simulink model "g1_centroidal_planner"  (R2025b)
settings: Solver=FixedStepDiscrete  StartTime=0.0  StopTime=0.05  FixedStep=0.002  RelTol=1e-3
model workspace (MAT data in the model file):
  accelerationKd = [0; 0; 0; 0; 0; 0; 0; 0; 0; 0; 0; 0; 0; 0; 0; 0; 0; 0; 0; 0; 0; 0; 0]
  accelerationKp = [0; 0; 0; 0; 0; 0; 0; 0; 0; 0; 0; 0; 0; 0; 0; 0; 0; 0; 0; 0; 0; 0; 0]
  g1_mpc_joint_indices = [4 5 6 7 1 2 17 18 19 20 14 15 29 28 27 8 9 10 3 21 22 23 16]
values from neighbouring files (symbols this model uses):
  g1_kd = 10.0 10.0 10.0 10.0 10.0 10.0 10.0 10.0 10.0 10.0 1.0 1.0 1.0 10.0 10.0 10.0 10.0 10.0 10.0 10.0 10.0 10.0 10.0 1.0 1.0 1.0 10.0 10.0 10.0    [g1_data.sldd]
  g1_kp = 1200.0 1200.0 1200.0 1200.0 1200.0 1200.0 1200.0 1200.0 1200.0 1200.0 100.0 100.0 100.0 1200.0 1200.0 1200.0 1200.0 1200.0 1200.0 1200.0 1200.0 1200.0 1200.0 100.0 100.0 100.0 1200.0 1200.0 1200.0    [g1_data.sldd]
  g1_mpc_to_plant = 0.0 0.0 0.0 1.0 0.0 0.0 0.0 0.0 0.0 0.0 0.0 0.0 0.0 0.0 0.0 0.0 0.0 0.0 0.0 0.0 0.0 0.0 0.0 0.0 0.0 0.0 0.0 0.0 0.0 0.0 0.0 0.0 0.0 1.0 0.0 0.0 0.0 0.0 0.0 0.0 0.0 0.0 0.0 0.0 0.0 0.0 0.0 0.0 0.0 0.0 0.0 0.0 0.0 0.0 0.0 0.0 0.0 0.0 0.0 0.0 0.0 0.0 0.0 1.0 0.0 0.0 0.0 0.0 0.0 0.0 0.0 0.0 0.0 0.0 0.0 0.0 0.0 0.0 0.0 0.0 0.0 0.0 0.0 0.0 0.0 0.0 0.0 0.0 0.0 0.0 0.0 0.0 0.0 1.0 0.0 0.0 0.0 0.0 0.0 0.0    [g1_data.sldd]
Description:
  | Centroidal synchronous MPC and policy query followed by independent inverse dynamics using measured q/v. Output: policy72, torque23, action95.
settings Model: DataDictionary=g1_data.sldd  Creator=enoch  LastModifiedBy=enoch

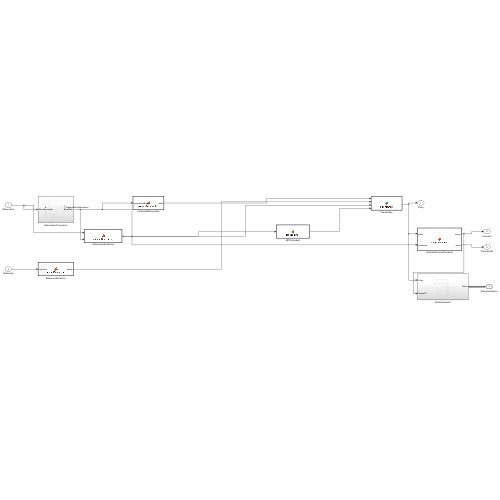
[thumbnail: Simulink's stored preview of the top-level diagram]
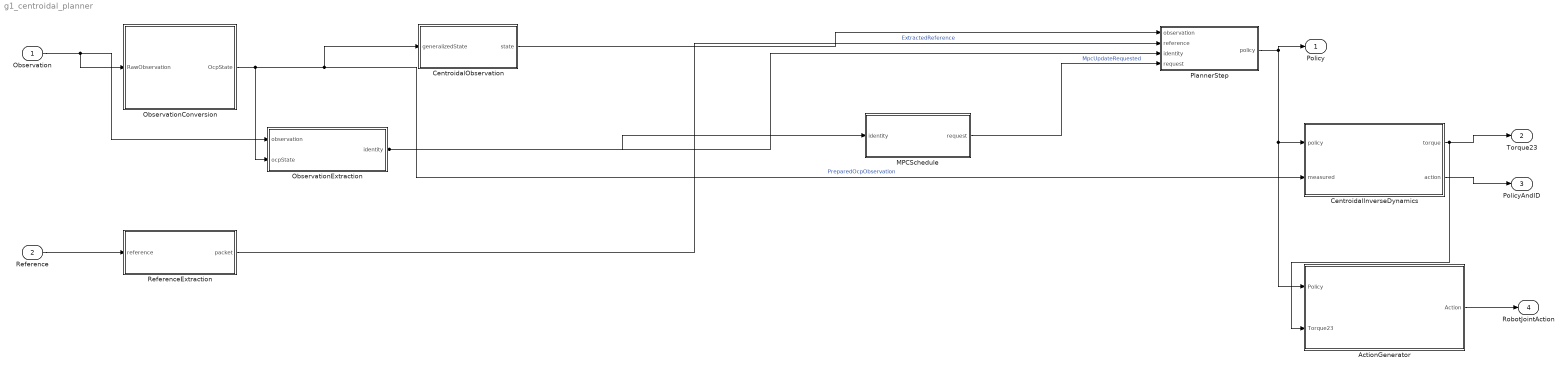
== system g1_centroidal_planner ==
  Observation : Inport  PortDimensions=74  SampleTime=0.002
  Reference : Inport  Port=2  PortDimensions=428  SampleTime=0.002
  ActionGenerator : Subsystem
  CentroidalInverseDynamics : MATLAB Function  TreatAsAtomicUnit=on
  CentroidalObservation : MATLAB Function  TreatAsAtomicUnit=on
  MPCSchedule : MATLAB Function  TreatAsAtomicUnit=on
  ObservationConversion : Subsystem
  ObservationExtraction : MATLAB Function  TreatAsAtomicUnit=on
  PlannerStep : MATLAB Function  TreatAsAtomicUnit=on
  ReferenceExtraction : MATLAB Function  TreatAsAtomicUnit=on
  Policy : Outport  PortDimensions=72
  Torque23 : Outport  Port=2  PortDimensions=23
  PolicyAndID : Outport  Port=3  PortDimensions=95
  RobotJointAction : Outport  Port=4  OutDataTypeStr=Bus: RobotJointAction
  wires:
  Observation/1 -> ObservationConversion/1(RawObservation), ObservationExtraction/1(observation)
  ObservationConversion/1(OcpState) -> CentroidalInverseDynamics/2(measured), CentroidalObservation/1(generalizedState), ObservationExtraction/2(ocpState)  "PreparedOcpObservation"
  Reference/1 -> ReferenceExtraction/1(reference)
  ReferenceExtraction/1(packet) -> PlannerStep/2(reference)  "ExtractedReference"
  CentroidalObservation/1(state) -> PlannerStep/1(observation)
  ObservationExtraction/1(identity) -> PlannerStep/3(identity), MPCSchedule/1(identity)
  MPCSchedule/1(request) -> PlannerStep/4(request)  "MpcUpdateRequested"
  PlannerStep/1(policy) -> Policy/1, ActionGenerator/1(Policy), CentroidalInverseDynamics/1(policy)
  CentroidalInverseDynamics/1(torque) -> Torque23/1, ActionGenerator/2(Torque23)
  CentroidalInverseDynamics/2(action) -> PolicyAndID/1
  ActionGenerator/1(Action) -> RobotJointAction/1

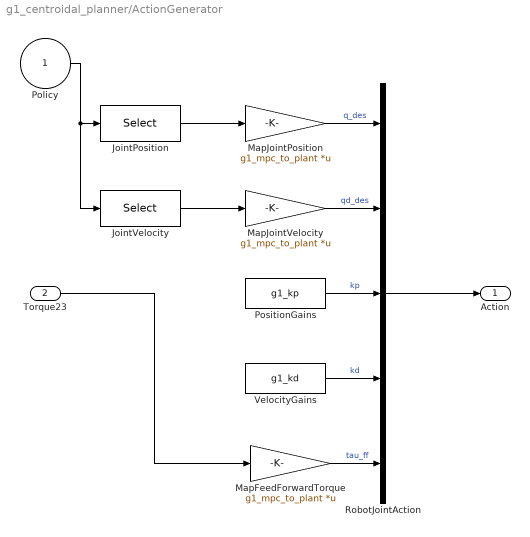
== system g1_centroidal_planner/ActionGenerator ==
  Policy : Inport  PortDimensions=72
  Torque23 : Inport  Port=2  PortDimensions=23
  JointPosition : Selector  InputPortWidth=72  IndexOptions=Index vector (dialog)  Indices=13:35  OutputSizes=1
  JointVelocity : Selector  InputPortWidth=72  IndexOptions=Index vector (dialog)  Indices=48:70  OutputSizes=1
  MapFeedForwardTorque : Gain  Gain=g1_mpc_to_plant  Multiplication=Matrix(K*u)
  MapJointPosition : Gain  Gain=g1_mpc_to_plant  Multiplication=Matrix(K*u)
  MapJointVelocity : Gain  Gain=g1_mpc_to_plant  Multiplication=Matrix(K*u)
  PositionGains : Constant  Value=g1_kp
  RobotJointAction : BusCreator  Inputs=5  OutDataTypeStr=Bus: RobotJointAction  NonVirtualBus=on
  VelocityGains : Constant  Value=g1_kd
  Action : Outport  OutDataTypeStr=Bus: RobotJointAction
  wires:
  MapJointPosition/1 -> RobotJointAction/1  "q_des"
  MapJointVelocity/1 -> RobotJointAction/2  "qd_des"
  PositionGains/1 -> RobotJointAction/3  "kp"
  VelocityGains/1 -> RobotJointAction/4  "kd"
  MapFeedForwardTorque/1 -> RobotJointAction/5  "tau_ff"
  RobotJointAction/1 -> Action/1
  Torque23/1 -> MapFeedForwardTorque/1
  JointVelocity/1 -> MapJointVelocity/1
  JointPosition/1 -> MapJointPosition/1
  Policy/1 -> JointVelocity/1, JointPosition/1

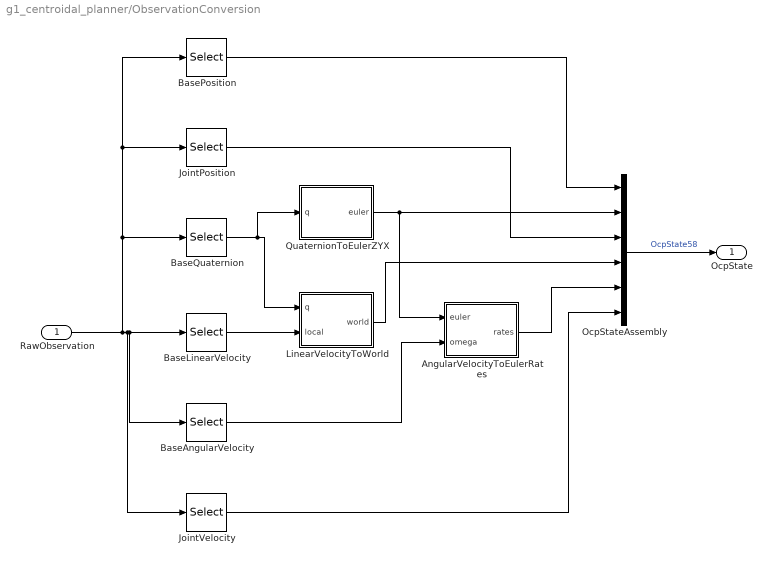
== system g1_centroidal_planner/ObservationConversion ==
  RawObservation : Inport
  AngularVelocityToEulerRates : MATLAB Function  TreatAsAtomicUnit=on
  BaseAngularVelocity : Selector  InputPortWidth=74  IndexOptions=Index vector (dialog)  Indices=12:14  OutputSizes=1
  BaseLinearVelocity : Selector  InputPortWidth=74  IndexOptions=Index vector (dialog)  Indices=9:11  OutputSizes=1
  BasePosition : Selector  InputPortWidth=74  IndexOptions=Index vector (dialog)  Indices=2:4  OutputSizes=1
  BaseQuaternion : Selector  InputPortWidth=74  IndexOptions=Index vector (dialog)  Indices=5:8  OutputSizes=1
  JointPosition : Selector  InputPortWidth=74  IndexOptions=Index vector (dialog)  Indices=14+g1_mpc_joint_indices  OutputSizes=1
  JointVelocity : Selector  InputPortWidth=74  IndexOptions=Index vector (dialog)  Indices=43+g1_mpc_joint_indices  OutputSizes=1
  LinearVelocityToWorld : MATLAB Function  TreatAsAtomicUnit=on
  OcpStateAssembly : Mux  Inputs=6
  QuaternionToEulerZYX : MATLAB Function  TreatAsAtomicUnit=on
  OcpState : Outport
  wires:
  RawObservation/1 -> BaseQuaternion/1, BasePosition/1, JointPosition/1, JointVelocity/1, BaseAngularVelocity/1, BaseLinearVelocity/1
  BaseQuaternion/1 -> LinearVelocityToWorld/1(q), QuaternionToEulerZYX/1(q)
  BasePosition/1 -> OcpStateAssembly/1
  JointPosition/1 -> OcpStateAssembly/3
  JointVelocity/1 -> OcpStateAssembly/6
  OcpStateAssembly/1 -> OcpState/1  "OcpState58"
  BaseLinearVelocity/1 -> LinearVelocityToWorld/2(local)
  QuaternionToEulerZYX/1(euler) -> OcpStateAssembly/2, AngularVelocityToEulerRates/1(euler)
  BaseAngularVelocity/1 -> AngularVelocityToEulerRates/2(omega)
  LinearVelocityToWorld/1(world) -> OcpStateAssembly/4
  AngularVelocityToEulerRates/1(rates) -> OcpStateAssembly/5

== matlab function g1_centroidal_planner/ObservationExtraction ==
  data: observation input; identity output; ocpState input; g1_mpc_joint_indices parameter
function identity = extractObservation(observation, ocpState, g1_mpc_joint_indices)
state=ocpState; indices=g1_mpc_joint_indices;
%EXTRACTOBSERVATION Check observation/state mapping and return tick identity.
%#codegen
% Derived from ObservationExtractionMex.cpp; see licenses/observation_conversion.txt.
assert(isa(observation,'double') && isreal(observation) && ~issparse(observation) && numel(observation)==74,'G1:ObservationExtraction','Invalid observation type or dimension');
assert(isa(state,'double') && isreal(state) && ~issparse(state) && numel(state)==58,'G1:ObservationExtraction','Invalid state type or dimension');
assert(isa(indices,'double') && isreal(indices) && ~issparse(indices) && numel(indices)==23,'G1:ObservationExtraction','Invalid joint index type or dimension');
assert(all(isfinite(observation(:))) && all(isfinite(state(:))),'G1:ObservationExtraction','Nonfinite observation or state');
t=observation(1);
assert(t>=0 && t/.002<=9007199254740992,'G1:ObservationExtraction','Invalid physical time');
tick=round(t/.002); canonical=tick*.002;
assert(abs(t-canonical)<=1e-12,'G1:ObservationExtraction','Raw time exceeds canonical tick tolerance');
assert(observation(4)>=.35 && observation(4)<=1.3,'G1:ObservationExtraction','Base height outside safety envelope');
q=observation(5:8);
pitch=asin(max(-1,min(1,2*(q(1)*q(3)-q(4)*q(2)))));
roll=atan2(2*(q(1)*q(2)+q(3)*q(4)),1-2*(q(2)*q(2)+q(3)*q(3)));
assert(abs(pitch)<=pi/4 && abs(roll)<=pi/4,'G1:ObservationExtraction','Tilt outside safety envelope');
assert(abs(norm(q)-1)<=1e-6,'G1:ObservationExtraction','Quaternion rejected');
for j=1:3
    assert(state(j)==observation(1+j),'G1:ObservationExtraction','OCP position identity mismatch');
end
seen=false(29,1);
for j=1:23
    k=indices(j);
    assert(isfinite(k) && k>=1 && k<=29 && k==floor(k),'G1:ObservationExtraction','Invalid joint index');
    assert(~seen(k),'G1:ObservationExtraction','Duplicate joint index');
    seen(k)=true;
    assert(state(6+j)==observation(14+k) && state(35+j)==observation(43+k),'G1:ObservationExtraction','OCP joint mapping mismatch');
end
identity=[tick;canonical;t];
end

== matlab function g1_centroidal_planner/MPCSchedule ==
  data: identity input; request output
function request = scheduleMpc(identity)
%#codegen
% Same physical-deadline rule as the accepted scheduler; never retime observation.
coder.extrinsic('g1.plannerMex');
persistent epoch nextSlot previousTick previousRequest period
if isempty(epoch)
    period=0;period=g1.plannerMex('mpc_period');
    epoch=identity(2);nextSlot=1;previousTick=identity(1);previousRequest=true;
    request=1;return
end
if identity(1)==previousTick
    request=double(previousRequest);return
end
assert(identity(1)==previousTick+1);
t=identity(2);deadline=epoch+nextSlot*period;
due=(t+1e-12>=deadline);
if due
    while epoch+(nextSlot+1)*period<=t+1e-12
        nextSlot=nextSlot+1;
    end
    nextSlot=nextSlot+1;
end
previousTick=identity(1);previousRequest=due;request=double(due);
end

== matlab function g1_centroidal_planner/PlannerStep ==
  data: observation input; policy output; reference input; identity input; request input
function policy=plannerStep(observation,reference,identity,request)
%#codegen
% 显式数据流：提交本步数据、可选求解、查询策略。
coder.extrinsic('g1.plannerMex');
policy=zeros(72,1);
policy=g1.plannerMex('step',observation,reference,identity,request);
end

== matlab function g1_centroidal_planner/CentroidalObservation ==
  data: generalizedState input; state output
function state = convertObservation(generalizedState)
%#codegen
% 用当前模型的 A(q)*v/m 得到世界系归一化质心动量。
% 后 29 项是基座位姿和 23 个关节角；不调用逆动力学。
coder.extrinsic('g1.plannerMex');
state=zeros(35,1);
state=g1.plannerMex('convert_observation',generalizedState);
end

== matlab function g1_centroidal_planner/ObservationConversion/QuaternionToEulerZYX ==
  data: q input; euler output
function euler = quaternionToEulerZYX(q)
%QUATERNIONTOEULERZYX Convert wxyz quaternion to [yaw; pitch; roll].
%#codegen
% Derived from ObservationMex.cpp; see licenses/observation_conversion.txt.
assert(isa(q,'double') && isreal(q) && ~issparse(q) && numel(q)==4);
assert(all(isfinite(q(:))));
w=q(1); x=q(2); y=q(3); z=q(4);
euler = [atan2(2*(w*z+x*y),1-2*(y*y+z*z)); ...
    asin(2*(w*y-z*x)); atan2(2*(w*x+y*z),1-2*(x*x+y*y))];
assert(isreal(euler) && all(isfinite(euler)));
end

== matlab function g1_centroidal_planner/ObservationConversion/LinearVelocityToWorld ==
  data: q input; world output; local input
function world = linearVelocityToWorld(q, local)
%ROTATELINEARVELOCITY Rotate local velocity into world using wxyz quaternion.
%#codegen
% Derived from ObservationMex.cpp; see licenses/observation_conversion.txt.
assert(isa(q,'double') && isreal(q) && ~issparse(q) && numel(q)==4);
assert(isa(local,'double') && isreal(local) && ~issparse(local) && numel(local)==3);
assert(all(isfinite(q(:))) && all(isfinite(local(:))));
% Same quaternion-vector identity as Eigen; do not normalize the quaternion.
v=local(:); xyz=q(2:4); xyz=xyz(:);
uv=2*cross(xyz,v);
world=v+q(1)*uv+cross(xyz,uv);
assert(all(isfinite(world)));
end

== matlab function g1_centroidal_planner/ObservationConversion/AngularVelocityToEulerRates ==
  data: euler input; rates output; omega input
function rates = angularVelocityToEulerRates(euler, omega)
%LOCALANGULARVELOCITYTOEULERRATES Local omega to [yaw; pitch; roll] rates.
%#codegen
% Derived from ObservationMex.cpp; see licenses/observation_conversion.txt.
assert(isa(euler,'double') && isreal(euler) && ~issparse(euler) && numel(euler)==3);
assert(isa(omega,'double') && isreal(omega) && ~issparse(omega) && numel(omega)==3);
assert(all(isfinite(euler(:))) && all(isfinite(omega(:))));
sy=sin(euler(2)); cy=cos(euler(2)); sx=sin(euler(3)); cx=cos(euler(3));
tmp=sx*omega(2)/cy+cx*omega(3)/cy;
rates=[tmp;cx*omega(2)-sx*omega(3);omega(1)+sy*tmp];
assert(all(isfinite(rates)));
end

== matlab function g1_centroidal_planner/ReferenceExtraction ==
  data: reference input; packet output
function packet=extractReference(reference)
%#codegen
% 总线中 58 项是完整运动学参考；在这里转换为 35 项质心状态。
coder.extrinsic('g1.plannerMex');
assert(numel(reference)==428 && all(isfinite(reference(:))));
packet=zeros(359,1);packet(1:6)=reference(1:6);
if reference(2)==0,return;end
assert(reference(3)==1 || reference(3)==3);
for k=0:reference(3)-1
  state=zeros(35,1);
  state=g1.plannerMex('convert_observation',reference(7+58*k:64+58*k));
  packet(7+35*k:41+35*k)=state;
end
packet(112:216)=reference(181:285);
packet(217:359)=reference(286:428);
end

== matlab function g1_centroidal_planner/CentroidalInverseDynamics ==
  data: policy input; torque output; measured input; action output; accelerationKp parameter; accelerationKd parameter
function [torque,action]=inverseDynamics(policy,measured,accelerationKp, accelerationKd)
%#codegen
% 策略末尾是关节速度；加速度由显式反馈参数给出，默认均为零。
% 逆动力学使用实测 q/v 和 MPC 接触力，不从零关节速度输入反推动量。
coder.extrinsic('g1.plannerMex');
qdd=accelerationKp.*(policy(13:35)-measured(7:29))+ ...
    accelerationKd.*(policy(48:70)-measured(36:58));
torque=zeros(23,1);
torque=g1.plannerMex('centroidal_inverse_dynamics',policy,measured,qdd);
action=[policy(1:70);torque;policy(71:72)];
end
